simulink model "nlmodel"  (R2025b)
settings: Solver=FixedStepAuto  StartTime=0.0  StopTime=10  FixedStep=1e-5  MaxStep=1e-5  RelTol=1e-5
model workspace (MAT data in the model file):
  op_trim1 = opcond.OperatingReport
  op_trim1.Outputs_(1) = opcond.OutputReport
  op_trim1.Outputs_(1).yspec_ = 0
  op_trim1.Outputs_(1).Block_ = 'nlmodel/yf'
  op_trim1.Outputs_(1).PortWidth_ = 1
  op_trim1.Outputs_(1).PortNumber_ = NaN
  op_trim1.Outputs_(1).y_ = -0.000308512479988
  op_trim1.Outputs_(1).Known_ = 0
  op_trim1.Outputs_(1).Min_ = -Inf
  op_trim1.Outputs_(1).Max_ = Inf
  op_trim1.Outputs_(2) = opcond.OutputReport
  op_trim1.Outputs_(2).yspec_ = 0
  op_trim1.Outputs_(2).Block_ = 'nlmodel/ym'
  op_trim1.Outputs_(2).PortWidth_ = 1
  op_trim1.Outputs_(2).PortNumber_ = NaN
  op_trim1.Outputs_(2).y_ = 0.000280578391297
  op_trim1.Outputs_(2).Known_ = 0
  op_trim1.Outputs_(2).Min_ = -Inf
  op_trim1.Outputs_(2).Max_ = Inf
  op_trim1.TerminationString_ = 'Operating point specifications were successfully met.'
  op_trim1.OptimizationOutput_.iterations = 2
  op_trim1.OptimizationOutput_.funcCount = 35
  op_trim1.OptimizationOutput_.lssteplength = 1
  op_trim1.OptimizationOutput_.stepsize = 3.10253532537e-08
  op_trim1.OptimizationOutput_.algorithm = 'active-set'
  op_trim1.OptimizationOutput_.firstorderopt = 3.08933880934e-07
  op_trim1.OptimizationOutput_.constrviolation = 4.93311988481e-17
  op_trim1.OptimizationOutput_.message = 'Local minimum found that satisfies the constraints.
    | 
    | Optimization completed because the objective function is non-decreasing in 
    | feasible directions, to within the value of the optimality tolerance,
    | and constraints are satisfied to within the  value of the constraint tolerance.
    | 
    | <stopping criteria details>
    | 
    | Optimization completed: The first-order optimality measure, 3.089339e-07, is less
    | than options.OptimalityTolerance = 1.000000e-06, and the maximum constraint violation,
    | 4.933120e-17,is less than options.ConstraintTolerance = 1.000000e-06.'
  op_trim1.OptimizationOutput_.bestfeasible.x = [0.000138848122245; 8.30517542493e-05; -0.000130504703728; 7.18387192426e-05; 0; 0; 0; 0; -0.000972462343051; 0.000970846359403]
  op_trim1.OptimizationOutput_.bestfeasible.fval = 0
  op_trim1.OptimizationOutput_.bestfeasible.constrviolation = 4.93311988481e-17
  op_trim1.OptimizationOutput_.bestfeasible.firstorderopt = 3.08933880934e-07
  op_trim1.OptimizationOutput_.progress = {'<font face="monospaced"; size=3><BR>', 'Optimizing to solve for all desired dx/dt=0, x(k+1)-x(k)=0, and y=ydes.<BR>', ' <BR>', '(Maximum Error)  Block<BR>', ' ---------------------------------------------------------<BR>', '(2.23955e+02) nlmodel/Subsystem/Integrator4<BR>', '(5.45298e-05) nlmodel/Subsystem/Integrator4<BR>', '(4.93312e-17) nlmodel/Subsystem/Integrator4<BR>', '(4.93312e-17) nlmodel/Subsystem/Integrator4<BR>', ' <BR>', 'Operating point specifications were successfully met.<BR>'}
  op_trim1.Model_ = 'nlmodel'
  op_trim1.States_(1) = opcond.StateReport
  op_trim1.States_(1).dx_ = 1.51788304148e-18
  op_trim1.States_(1).Nx_ = 1
  op_trim1.States_(1).Block_ = 'nlmodel/Subsystem/Integrator'
  op_trim1.States_(1).SteadyState_ = 1
  op_trim1.States_(1).dxMin_ = -Inf
  op_trim1.States_(1).dxMax_ = Inf
  op_trim1.States_(1).Known_ = 0
  op_trim1.States_(1).Min_ = -Inf
  op_trim1.States_(1).Max_ = Inf
  op_trim1.States_(2) = opcond.StateReport
  op_trim1.States_(2).Nx_ = 1
  op_trim1.States_(2).Block_ = 'nlmodel/Subsystem/Integrator1'
  op_trim1.States_(2).x_ = 8.30517542493e-05
  op_trim1.States_(2).SteadyState_ = 1
  op_trim1.States_(2).dxMin_ = -Inf
  op_trim1.States_(2).dxMax_ = Inf
  op_trim1.States_(2).Known_ = 0
  op_trim1.States_(2).Min_ = -Inf
  op_trim1.States_(2).Max_ = Inf
  op_trim1.States_(3) = opcond.StateReport
  op_trim1.States_(3).dx_ = 4.33680868994e-19
  op_trim1.States_(3).Nx_ = 1
  op_trim1.States_(3).Block_ = 'nlmodel/Subsystem/Integrator2'
  op_trim1.States_(3).SteadyState_ = 1
  op_trim1.States_(3).dxMin_ = -Inf
  op_trim1.States_(3).dxMax_ = Inf
  op_trim1.States_(3).Known_ = 0
  op_trim1.States_(3).Min_ = -Inf
  op_trim1.States_(3).Max_ = Inf
  op_trim1.States_(4) = opcond.StateReport
  op_trim1.States_(4).Nx_ = 1
  op_trim1.States_(4).Block_ = 'nlmodel/Subsystem/Integrator3'
  op_trim1.States_(4).x_ = 0.000138848122245
  op_trim1.States_(4).SteadyState_ = 1
  op_trim1.States_(4).dxMin_ = -Inf
  op_trim1.States_(4).dxMax_ = Inf
  op_trim1.States_(4).Known_ = 0
  op_trim1.States_(4).Min_ = -Inf
  op_trim1.States_(4).Max_ = Inf
  op_trim1.States_(5) = opcond.StateReport
  op_trim1.States_(5).dx_ = -4.93311988481e-17
  op_trim1.States_(5).Nx_ = 1
  op_trim1.States_(5).Block_ = 'nlmodel/Subsystem/Integrator4'
  op_trim1.States_(5).SteadyState_ = 1
  op_trim1.States_(5).dxMin_ = -Inf
  op_trim1.States_(5).dxMax_ = Inf
  op_trim1.States_(5).Known_ = 0
  op_trim1.States_(5).Min_ = -Inf
  op_trim1.States_(5).Max_ = Inf
  op_trim1.States_(6) = opcond.StateReport
  op_trim1.States_(6).Nx_ = 1
  op_trim1.States_(6).Block_ = 'nlmodel/Subsystem/Integrator5'
  op_trim1.States_(6).x_ = -0.000130504703728
  op_trim1.States_(6).SteadyState_ = 1
  op_trim1.States_(6).dxMin_ = -Inf
  op_trim1.States_(6).dxMax_ = Inf
  op_trim1.States_(6).Known_ = 0
  op_trim1.States_(6).Min_ = -Inf
  op_trim1.States_(6).Max_ = Inf
  op_trim1.States_(7) = opcond.StateReport
  op_trim1.States_(7).dx_ = -4.55364912444e-17
  op_trim1.States_(7).Nx_ = 1
  op_trim1.States_(7).Block_ = 'nlmodel/Subsystem/Integrator6'
  op_trim1.States_(7).SteadyState_ = 1
  op_trim1.States_(7).dxMin_ = -Inf
  op_trim1.States_(7).dxMax_ = Inf
  op_trim1.States_(7).Known_ = 0
  op_trim1.States_(7).Min_ = -Inf
  op_trim1.States_(7).Max_ = Inf
  op_trim1.States_(8) = opcond.StateReport
  op_trim1.States_(8).Nx_ = 1
  op_trim1.States_(8).Block_ = 'nlmodel/Subsystem/Integrator7'
  op_trim1.States_(8).x_ = 7.18387192426e-05
  op_trim1.States_(8).SteadyState_ = 1
  op_trim1.States_(8).dxMin_ = -Inf
  op_trim1.States_(8).dxMax_ = Inf
  op_trim1.States_(8).Known_ = 0
  op_trim1.States_(8).Min_ = -Inf
  op_trim1.States_(8).Max_ = Inf
  op_trim1.Inputs_(1) = opcond.InputReport
  op_trim1.Inputs_(1).Block_ = 'nlmodel/uf'
  op_trim1.Inputs_(1).PortWidth_ = 1
  op_trim1.Inputs_(1).PortDimensions_ = [1 1]
  op_trim1.Inputs_(1).u_ = -0.000972462343051
  op_trim1.Inputs_(1).Known_ = 0
  op_trim1.Inputs_(1).Min_ = -Inf
  op_trim1.Inputs_(1).Max_ = Inf
  op_trim1.Inputs_(2) = opcond.InputReport
  op_trim1.Inputs_(2).Block_ = 'nlmodel/um'
  op_trim1.Inputs_(2).PortWidth_ = 1
  op_trim1.Inputs_(2).PortDimensions_ = [1 1]
  op_trim1.Inputs_(2).u_ = 0.000970846359403
  op_trim1.Inputs_(2).Known_ = 0
  op_trim1.Inputs_(2).Min_ = -Inf
  op_trim1.Inputs_(2).Max_ = Inf
undefined symbols (not defined in the file): activate_noise, dphi_0, dza_0, dzf_0, dzm_0, K, noise, params, phi_0, za_0, zf_0, zm_0
settings Model: Creator=pasqualederosa  LastModifiedBy=pasqualederosa
settings SolverCC: EnableFixedStepZeroCrossing=on
settings DataIOCC: ExternalInput=getinputstruct(op_trim1)  InitialState=getstatestruct(op_trim1)

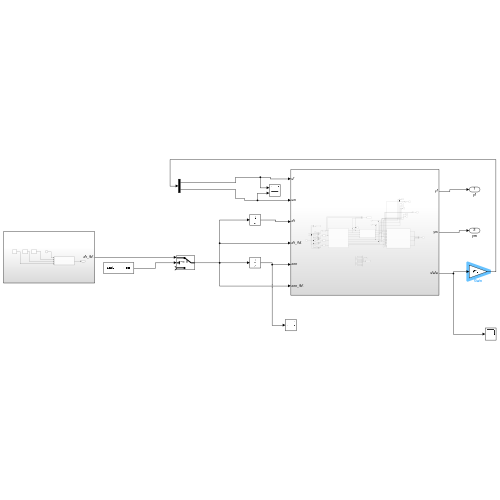
[thumbnail: Simulink's stored preview of the top-level diagram]
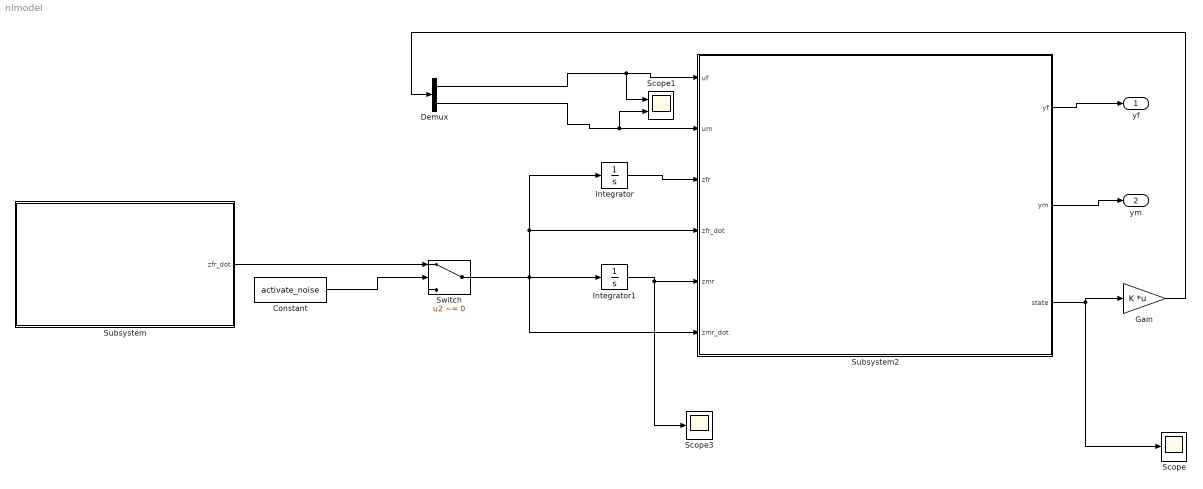
== system nlmodel ==
  Constant : Constant  Value=activate_noise
  Demux : Demux  Outputs=2
  Gain : Gain  Gain=K  Multiplication=Matrix(K*u)
  Integrator : Integrator
  Integrator1 : Integrator
  Scope : Scope
      settings: ActiveDisplayYMinimum=-0.53156363115471983  ActiveDisplayYMaximum=0.91717012850913848
  Scope1 : Scope  NumInputPorts=2
      settings: ActiveDisplayYMinimum=-142095.59925459951  ActiveDisplayYMaximum=71041.7943141915
  Scope3 : Scope
      settings: ActiveDisplayYMinimum=0.00820664752267481  ActiveDisplayYMaximum=0.063063941155904579  DataLoggingVariableName=ScopeData5
  Subsystem : Subsystem
  Subsystem2 : Subsystem
  Switch : Switch  Criteria=u2 ~= 0  SaturateOnIntegerOverflow=off  InputSameDT=off
  yf : Outport
  ym : Outport  Port=2
  wires:
  Subsystem2/1(yf) -> yf/1
  Subsystem2/2(ym) -> ym/1
  Switch/1 -> Subsystem2/6(zmr_dot), Integrator/1, Subsystem2/4(zfr_dot), Integrator1/1
  Integrator1/1 -> Scope3/1, Subsystem2/5(zmr)
  Integrator/1 -> Subsystem2/3(zfr)
  Subsystem2/3(state) -> Gain/1, Scope/1
  Gain/1 -> Demux/1
  Demux/1 -> Scope1/1, Subsystem2/1(uf)
  Demux/2 -> Scope1/2, Subsystem2/2(um)
  Subsystem/1(zfr_dot) -> Switch/1
  Constant/1 -> Switch/2

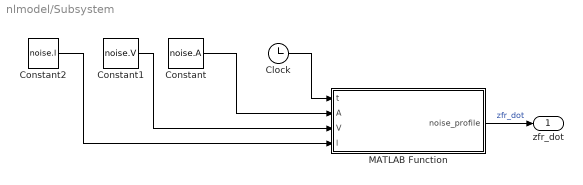
== system nlmodel/Subsystem ==
  Clock : Clock
  Constant : Constant  Value=noise.A
  Constant1 : Constant  Value=noise.V
  Constant2 : Constant  Value=noise.l
  MATLAB Function : MATLAB Function  TreatAsAtomicUnit=on
  zfr_dot : Outport
  wires:
  MATLAB Function/1(noise_profile) -> zfr_dot/1  "zfr_dot"
  Constant/1 -> MATLAB Function/2(A)
  Constant1/1 -> MATLAB Function/3(V)
  Constant2/1 -> MATLAB Function/4(l)
  Clock/1 -> MATLAB Function/1(t)

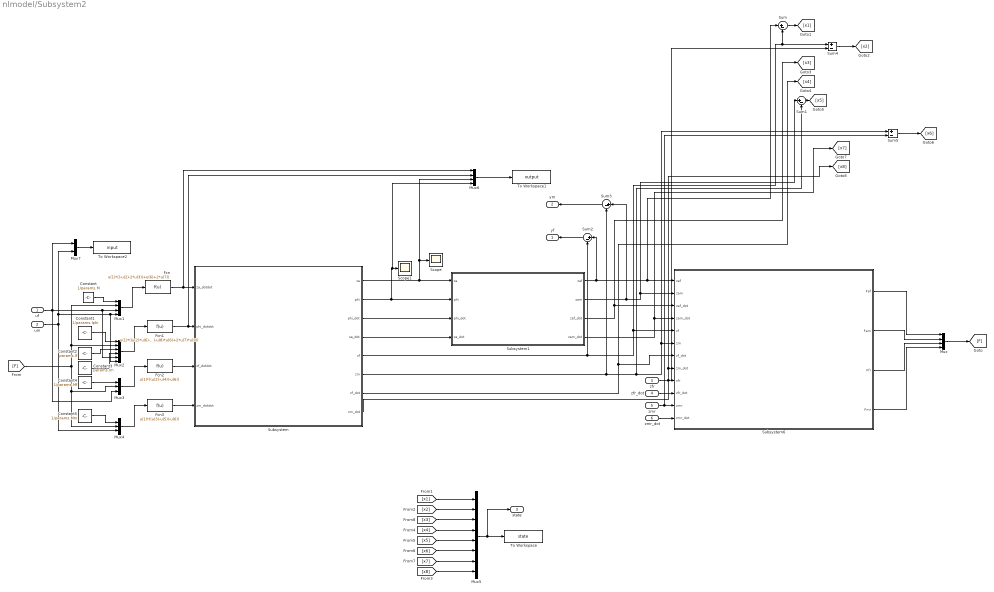
== system nlmodel/Subsystem2 ==
  uf : Inport
  um : Inport  Port=2
  zfr : Inport  Port=3
  zfr_dot : Inport  Port=4
  zmr : Inport  Port=5
  zmr_dot : Inport  Port=6
  Constant : Constant  Value=1/params.M
  Constant1 : Constant  Value=1/params.Iphi
  Constant2 : Constant  Value=params.lf
  Constant3 : Constant  Value=params.lm
  Constant4 : Constant  Value=1/params.Mf
  Constant5 : Constant  Value=1/params.Mm
  Fcn : Fcn  Expr=u(1)*((-u(2)-2*u(3))+u(6)+2*u(7))
  Fcn1 : Fcn  Expr=u(1)*((u(2)*u(6)-2*u(3)*u(7))-u(8)*u(6)+2*u(7)*u(9))
  Fcn2 : Fcn  Expr=u(1)*((u(2)-u(4))-u(6))
  Fcn3 : Fcn  Expr=u(1)*((u(3)-u(5))-u(6))
  Mux : Mux
  Mux1 : Mux
  Mux2 : Mux  Inputs=6
  Mux3 : Mux  Inputs=3
  Mux4 : Mux  Inputs=3
  Mux5 : Mux  Inputs=8
  Mux6 : Mux
  Mux7 : Mux  Inputs=2
  Scope : Scope
      settings: ActiveDisplayYMinimum=-0.035821552952841285  ActiveDisplayYMaximum=0.095635281779023584  DataLoggingVariableName=ScopeData3
  Scope1 : Scope
      settings: ActiveDisplayYMinimum=-0.051861364363464418  ActiveDisplayYMaximum=0.0057623671742010624  DataLoggingVariableName=ScopeData4
  Subsystem : Subsystem
  Subsystem1 : Subsystem
  Subsystem6 : Subsystem
  Sum{,1..3} (4 alike) : Sum  Inputs=|+-
  Sum4 : Sum  Inputs=+-
  Sum5 : Sum  Inputs=+-
  To Workspace : ToWorkspace  VariableName=state  SaveFormat=Timeseries  SampleTime=-1
  To Workspace1 : ToWorkspace  VariableName=output  SaveFormat=Timeseries  SampleTime=-1
  To Workspace2 : ToWorkspace  VariableName=input  SaveFormat=Timeseries  SampleTime=-1
  yf : Outport
  ym : Outport  Port=2
  state : Outport  Port=3
  wires:
  Fcn/1 -> Subsystem/1(za_dotdot), Mux6/1
  Sum1/1 -> [x5]
  Constant1/1 -> Mux2/1
  [x6] -> Mux5/6
  Fcn2/1 -> Subsystem/3(zf_dotdot)
  Subsystem6/3(Ffr) -> Mux/3
  [x7] -> Mux5/7
  [x5] -> Mux5/5
  Subsystem6/1(Faf) -> Mux/1
  Mux4/1 -> Fcn3/1
  Constant/1 -> Mux1/1
  Mux1/1 -> Fcn/1
  Constant5/1 -> Mux4/1
  Subsystem/3(phi_dot) -> Subsystem1/3(phi_dot)
  Constant2/1 -> Mux2/3
  Sum/1 -> [x1]
  Mux5/1 -> state/1, To Workspace/1
  Constant3/1 -> Mux2/4
  Sum2/1 -> yf/1
  Constant4/1 -> Mux3/1
  Subsystem1/3(zaf_dot) -> Subsystem6/3(zaf_dot), [x3]
  Subsystem6/2(Fam) -> Mux/2
  [x8] -> Mux5/8
  um/1 -> Mux4/3, Mux7/2, Mux2/6, Mux1/4
  uf/1 -> Mux7/1, Mux2/5, Mux1/3, Mux3/3
  Mux/1 -> [F]
  Subsystem/4(za_dot) -> Subsystem1/4(za_dot)
  Mux2/1 -> Fcn1/1
  [x4] -> Mux5/4
  Subsystem/1(za) -> Scope/1, Mux6/3, Subsystem1/1(za)
  Subsystem1/2(zam) -> Sum3/1, Sum1/1, Subsystem6/2(zam)
  [x3] -> Mux5/3
  [F] -> Mux3/2, Mux4/2, Mux2/2, Mux1/2
  Subsystem/7(zf_dot) -> Subsystem6/7(zf_dot), [x4]
  Subsystem/5(zf) -> Sum2/2, Subsystem6/5(zf), Sum4/1, Sum/2
  [x2] -> Mux5/2
  Fcn1/1 -> Mux6/2, Subsystem/2(phi_dotdot)
  Subsystem6/4(Fmr) -> Mux/4
  Mux3/1 -> Fcn2/1
  Subsystem/6(zm) -> Sum5/1, Subsystem6/6(zm), Sum1/2, Sum3/2
  Subsystem1/1(zaf) -> Sum2/1, Sum/1, Subsystem6/1(zaf)
  [x1] -> Mux5/1
  Fcn3/1 -> Subsystem/4(zm_dotdot)
  Sum3/1 -> ym/1
  Subsystem/8(zm_dot) -> [x8], Subsystem6/8(zm_dot)
  Subsystem1/4(zam_dot) -> Subsystem6/4(zam_dot), [x7]
  zfr/1 -> Sum4/2, Subsystem6/9(zfr)
  zfr_dot/1 -> Subsystem6/10(zfr_dot)
  zmr/1 -> Subsystem6/11(zmr), Sum5/2
  zmr_dot/1 -> Subsystem6/12(zmr_dot)
  Sum4/1 -> [x2]
  Sum5/1 -> [x6]
  Subsystem/2(phi) -> Mux6/4, Scope1/1, Subsystem1/2(phi)
  Mux6/1 -> To Workspace1/1
  Mux7/1 -> To Workspace2/1

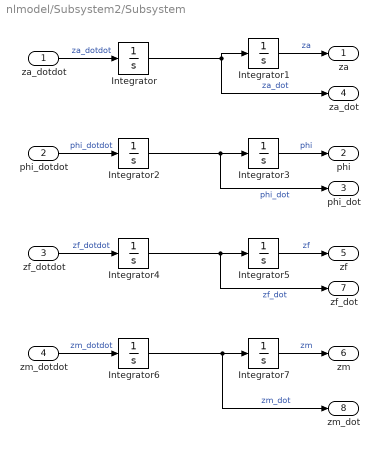
== system nlmodel/Subsystem2/Subsystem ==
  za_dotdot : Inport
  phi_dotdot : Inport  Port=2
  zf_dotdot : Inport  Port=3
  zm_dotdot : Inport  Port=4
  Integrator : Integrator  InitialCondition=dza_0
  Integrator1 : Integrator  InitialCondition=za_0
  Integrator2 : Integrator  InitialCondition=dphi_0
  Integrator3 : Integrator  InitialCondition=phi_0
  Integrator4 : Integrator  InitialCondition=dzf_0
  Integrator5 : Integrator  InitialCondition=zf_0
  Integrator6 : Integrator  InitialCondition=dzm_0
  Integrator7 : Integrator  InitialCondition=zm_0
  za : Outport
  phi : Outport  Port=2
  phi_dot : Outport  Port=3
  za_dot : Outport  Port=4
  zf : Outport  Port=5
  zm : Outport  Port=6
  zf_dot : Outport  Port=7
  zm_dot : Outport  Port=8
  wires:
  zm_dotdot/1 -> Integrator6/1  "zm_dotdot"
  Integrator7/1 -> zm/1  "zm"
  Integrator6/1 -> zm_dot/1, Integrator7/1  "zm_dot"
  Integrator3/1 -> phi/1  "phi"
  Integrator5/1 -> zf/1  "zf"
  Integrator1/1 -> za/1  "za"
  zf_dotdot/1 -> Integrator4/1  "zf_dotdot"
  Integrator2/1 -> phi_dot/1, Integrator3/1  "phi_dot"
  Integrator/1 -> Integrator1/1, za_dot/1  "za_dot"
  za_dotdot/1 -> Integrator/1  "za_dotdot"
  phi_dotdot/1 -> Integrator2/1  "phi_dotdot"
  Integrator4/1 -> zf_dot/1, Integrator5/1  "zf_dot"

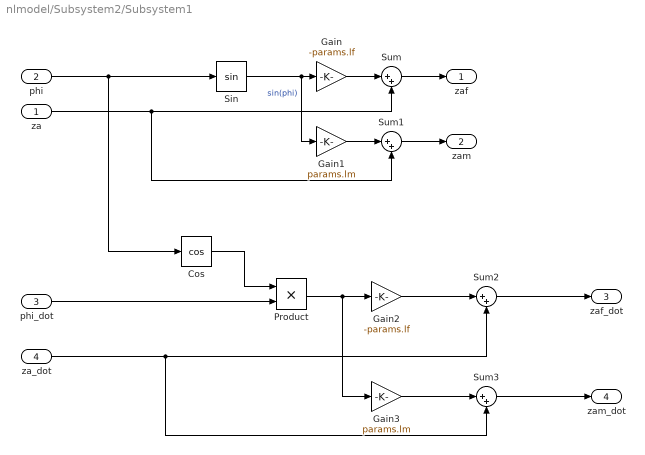
== system nlmodel/Subsystem2/Subsystem1 ==
  za : Inport
  phi : Inport  Port=2
  phi_dot : Inport  Port=3
  za_dot : Inport  Port=4
  Cos : Trigonometry  Operator=cos
  Gain : Gain  Gain=-params.lf
  Gain1 : Gain  Gain=params.lm
  Gain2 : Gain  Gain=-params.lf
  Gain3 : Gain  Gain=params.lm
  Product : Product
  Sin : Trigonometry
  Sum{,1..3} (4 alike) : Sum  Inputs=|++
  zaf : Outport
  zam : Outport  Port=2
  zaf_dot : Outport  Port=3
  zam_dot : Outport  Port=4
  wires:
  za/1 -> Sum1/2, Sum/2
  Gain/1 -> Sum/1
  phi/1 -> Cos/1, Sin/1
  Sum/1 -> zaf/1
  Sin/1 -> Gain1/1, Gain/1  "sin(phi)"
  Gain1/1 -> Sum1/1
  Sum1/1 -> zam/1
  Cos/1 -> Product/1
  phi_dot/1 -> Product/2
  Product/1 -> Gain2/1, Gain3/1
  Gain2/1 -> Sum2/1
  za_dot/1 -> Sum3/2, Sum2/2
  Sum2/1 -> zaf_dot/1
  Gain3/1 -> Sum3/1
  Sum3/1 -> zam_dot/1

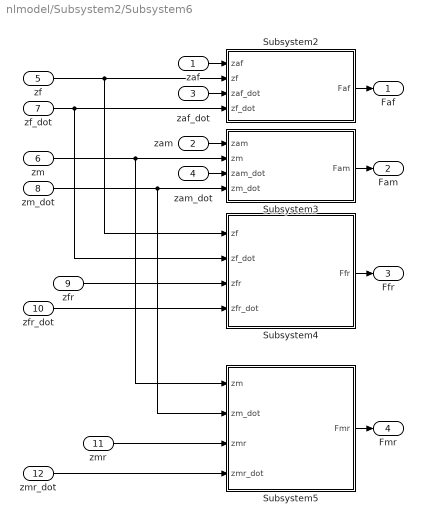
== system nlmodel/Subsystem2/Subsystem6 ==
  zaf : Inport
  zam : Inport  Port=2
  zaf_dot : Inport  Port=3
  zam_dot : Inport  Port=4
  zf : Inport  Port=5
  zm : Inport  Port=6
  zf_dot : Inport  Port=7
  zm_dot : Inport  Port=8
  zfr : Inport  Port=9
  zfr_dot : Inport  Port=10
  zmr : Inport  Port=11
  zmr_dot : Inport  Port=12
  Subsystem2 : Subsystem
  Subsystem3 : Subsystem
  Subsystem4 : Subsystem
  Subsystem5 : Subsystem
  Faf : Outport
  Fam : Outport  Port=2
  Ffr : Outport  Port=3
  Fmr : Outport  Port=4
  wires:
  zm_dot/1 -> Subsystem5/2(zm_dot), Subsystem3/4(zm_dot)
  zaf/1 -> Subsystem2/1(zaf)
  Subsystem2/1(Faf) -> Faf/1
  zam_dot/1 -> Subsystem3/3(zam_dot)
  zaf_dot/1 -> Subsystem2/3(zaf_dot)
  Subsystem3/1(Fam) -> Fam/1
  zf/1 -> Subsystem4/1(zf), Subsystem2/2(zf)
  Subsystem4/1(Ffr) -> Ffr/1
  Subsystem5/1(Fmr) -> Fmr/1
  zf_dot/1 -> Subsystem4/2(zf_dot), Subsystem2/4(zf_dot)
  zam/1 -> Subsystem3/1(zam)
  zm/1 -> Subsystem5/1(zm), Subsystem3/2(zm)
  zfr/1 -> Subsystem4/3(zfr)
  zfr_dot/1 -> Subsystem4/4(zfr_dot)
  zmr/1 -> Subsystem5/3(zmr)
  zmr_dot/1 -> Subsystem5/4(zmr_dot)

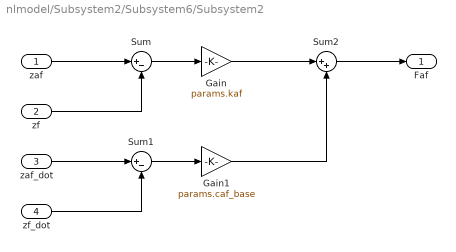
== system nlmodel/Subsystem2/Subsystem6/Subsystem2 ==
  zaf : Inport
  zf : Inport  Port=2
  zaf_dot : Inport  Port=3
  zf_dot : Inport  Port=4
  Gain : Gain  Gain=params.kaf
  Gain1 : Gain  Gain=params.caf_base
  Sum : Sum  Inputs=|+-
  Sum1 : Sum  Inputs=|+-
  Sum2 : Sum  Inputs=|++
  Faf : Outport
  wires:
  zaf/1 -> Sum/1
  zf/1 -> Sum/2
  zaf_dot/1 -> Sum1/1
  zf_dot/1 -> Sum1/2
  Sum/1 -> Gain/1
  Sum1/1 -> Gain1/1
  Gain/1 -> Sum2/1
  Gain1/1 -> Sum2/2
  Sum2/1 -> Faf/1

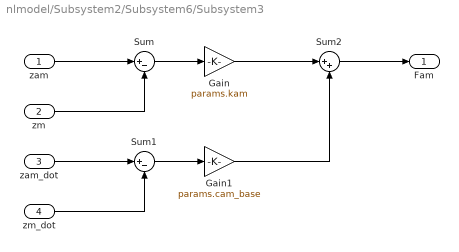
== system nlmodel/Subsystem2/Subsystem6/Subsystem3 ==
  zam : Inport
  zm : Inport  Port=2
  zam_dot : Inport  Port=3
  zm_dot : Inport  Port=4
  Gain : Gain  Gain=params.kam
  Gain1 : Gain  Gain=params.cam_base
  Sum : Sum  Inputs=|+-
  Sum1 : Sum  Inputs=|+-
  Sum2 : Sum  Inputs=|++
  Fam : Outport
  wires:
  zam/1 -> Sum/1
  zm/1 -> Sum/2
  zam_dot/1 -> Sum1/1
  zm_dot/1 -> Sum1/2
  Sum/1 -> Gain/1
  Sum1/1 -> Gain1/1
  Gain/1 -> Sum2/1
  Gain1/1 -> Sum2/2
  Sum2/1 -> Fam/1

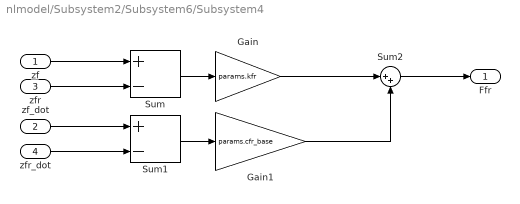
== system nlmodel/Subsystem2/Subsystem6/Subsystem4 ==
  zf : Inport
  zf_dot : Inport  Port=2
  zfr : Inport  Port=3
  zfr_dot : Inport  Port=4
  Gain : Gain  Gain=params.kfr
  Gain1 : Gain  Gain=params.cfr_base
  Sum : Sum  Inputs=+-
  Sum1 : Sum  Inputs=+-
  Sum2 : Sum  Inputs=|++
  Ffr : Outport
  wires:
  Gain/1 -> Sum2/1
  Sum2/1 -> Ffr/1
  Gain1/1 -> Sum2/2
  Sum/1 -> Gain/1
  zfr/1 -> Sum/2
  zf/1 -> Sum/1
  Sum1/1 -> Gain1/1
  zf_dot/1 -> Sum1/1
  zfr_dot/1 -> Sum1/2

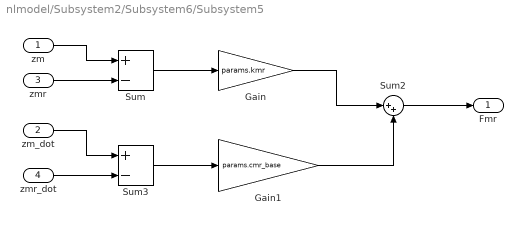
== system nlmodel/Subsystem2/Subsystem6/Subsystem5 ==
  zm : Inport
  zm_dot : Inport  Port=2
  zmr : Inport  Port=3
  zmr_dot : Inport  Port=4
  Gain : Gain  Gain=params.kmr
  Gain1 : Gain  Gain=params.cmr_base
  Sum : Sum  Inputs=+-
  Sum2 : Sum  Inputs=|++
  Sum3 : Sum  Inputs=+-
  Fmr : Outport
  wires:
  Gain/1 -> Sum2/1
  Sum2/1 -> Fmr/1
  Gain1/1 -> Sum2/2
  Sum3/1 -> Gain1/1
  Sum/1 -> Gain/1
  zm/1 -> Sum/1
  zmr/1 -> Sum/2
  zm_dot/1 -> Sum3/1
  zmr_dot/1 -> Sum3/2

== matlab function nlmodel/Subsystem/MATLAB Function ==
  data: t input; noise_profile output; A input; V input; l input
function noise_profile = calc_noise(t, A, V, l)
    % Delay start by 3 seconds
    delay = 3;
    
    if t < delay
        noise_profile = 0;
    elseif t > (l / V) + delay
        noise_profile = 0;
    else
        % Shift time by the delay so the equation evaluates from t=0
        t_shifted = t - delay;
        noise_profile = (A / 2) * (1 - cos((2 * pi * V / l) * t_shifted));
    end
end
